simulink model "plant_model_with_dither_input"  (R2024b)
settings: Solver=FixedStepAuto  StartTime=0.0  StopTime=60  FixedStep=T_sample  RelTol=1e-3
values from neighbouring files (symbols this model uses):
  T_sample = 0.01    [LS_demo_ident.m]    (also in P_ident.m)
libraries: simulink x1
settings Model: Creator=Kang  LastModifiedBy=sk3547969879
settings SolverCC: AlgebraicLoopSolver=TrustRegion
settings DebuggingCC: UnconnectedInputMsg=warning  UnconnectedOutputMsg=warning  UnconnectedLineMsg=warning
settings ModelReferenceCC: EnableRefExpFcnMdlSchedulingChecks=on
settings RTWCC: GPUComputeCapability=3.5  DLArmComputeVersion=19.05

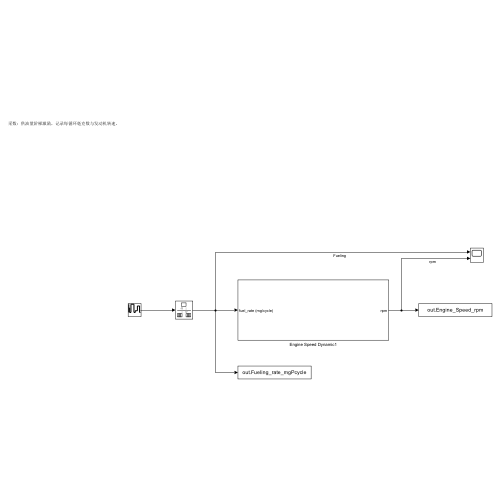
[thumbnail: Simulink's stored preview of the top-level diagram]
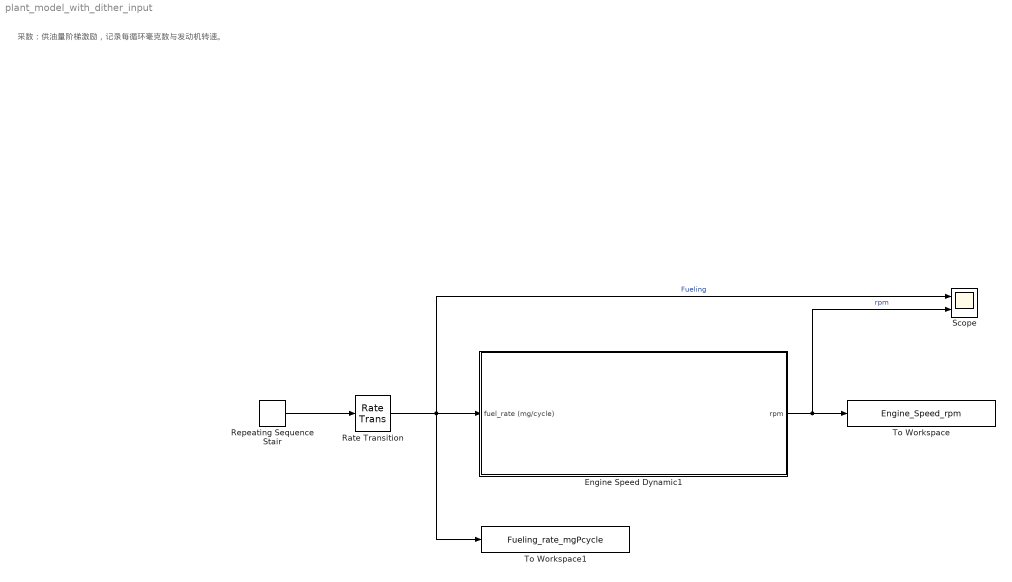
== system plant_model_with_dither_input ==
  note: 采数：供油量阶梯激励，记录每循环毫克数与发动机转速。
  Engine Speed Dynamic1 : Subsystem
  Rate Transition : RateTransition  InitialCondition=10
  Repeating Sequence Stair : simulink/Sources/Repeating Sequence Stair  OutValues=[15 10 20 20 20 10 12 12 18 18 10].'  tsamp=5  OutMin=[]  OutMax=[]  OutDataTypeStr=double  OutputDataTypeScalingMode=double  OutDataType=fixdt(0,8)  ConRadixGroup=Best Precision: Vector-wise  OutScaling=2^-12
  Scope : Scope  NumInputPorts=2
  To Workspace : ToWorkspace  VariableName=Engine_Speed_rpm  SaveFormat=Timeseries  SampleTime=T_sample
  To Workspace1 : ToWorkspace  VariableName=Fueling_rate_mgPcycle  SaveFormat=Timeseries  SampleTime=T_sample
  wires:
  Engine Speed Dynamic1/1(rpm) -> Scope/2, To Workspace/1  "rpm"
  Repeating Sequence Stair/1 -> Rate Transition/1
  Rate Transition/1 -> To Workspace1/1, Scope/1, Engine Speed Dynamic1/1(fuel_rate (mg/cycle))  "Fueling"

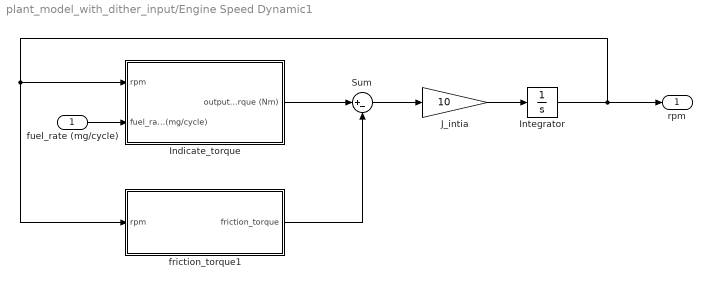
== system plant_model_with_dither_input/Engine Speed Dynamic1 ==
  fuel_rate (mg/cycle) : Inport
  Indicate_torque : Subsystem
  Integrator : Integrator  InitialCondition=960
  J_intia : Gain  Gain=10
  Sum : Sum  Inputs=|+-
  friction_torque1 : Subsystem
  rpm : Outport
  wires:
  Sum/1 -> J_intia/1
  Indicate_torque/1(output_torque (Nm)) -> Sum/1
  Integrator/1 -> rpm/1, friction_torque1/1(rpm), Indicate_torque/1(rpm)
  fuel_rate (mg/cycle)/1 -> Indicate_torque/2(fuel_rate (mg/cycle))
  friction_torque1/1(friction_torque) -> Sum/2
  J_intia/1 -> Integrator/1

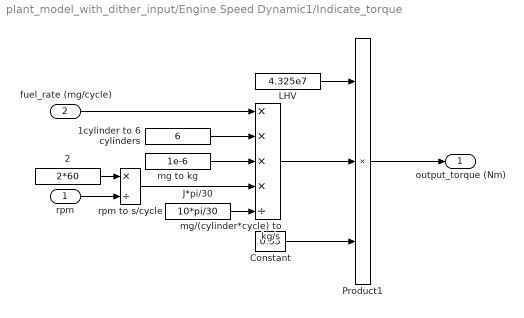
== system plant_model_with_dither_input/Engine Speed Dynamic1/Indicate_torque ==
  rpm : Inport
  fuel_rate (mg/cycle) : Inport  Port=2
  1cylinder to 6 cylinders : Constant  Value=6
  2 : Constant  Value=2*60
  Constant : Constant  Value=0.35
  J*pi/30 : Constant  Value=10*pi/30
  LHV : Constant  Value=4.325e7
  Product1 : Product  Inputs=3
  mg to kg : Constant  Value=1e-6
  mg/(cylinder*cycle) to kg/s : Product  Inputs=****/
  rpm to s/cycle : Product  Inputs=*/
  output_torque (Nm) : Outport
  wires:
  Product1/1 -> output_torque (Nm)/1
  Constant/1 -> Product1/3
  fuel_rate (mg/cycle)/1 -> mg/(cylinder*cycle) to kg/s/1
  1cylinder to 6 cylinders/1 -> mg/(cylinder*cycle) to kg/s/2
  2/1 -> rpm to s/cycle/1
  mg to kg/1 -> mg/(cylinder*cycle) to kg/s/3
  LHV/1 -> Product1/1
  J*pi/30/1 -> mg/(cylinder*cycle) to kg/s/5
  rpm to s/cycle/1 -> mg/(cylinder*cycle) to kg/s/4
  rpm/1 -> rpm to s/cycle/2
  mg/(cylinder*cycle) to kg/s/1 -> Product1/2

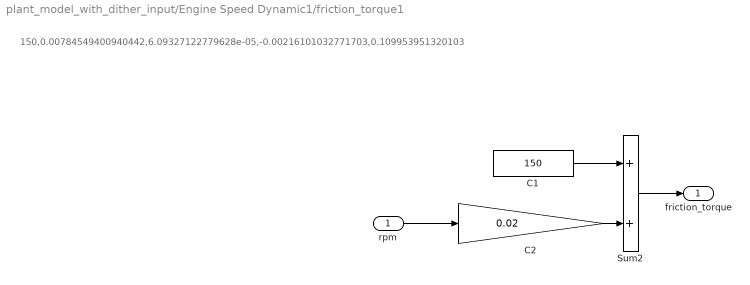
== system plant_model_with_dither_input/Engine Speed Dynamic1/friction_torque1 ==
  note: 150,0.00784549400940442,6.09327122779628e-05,-0.00216101032771703,0.109953951320103
  rpm : Inport
  C1 : Constant  Value=150
  C2 : Gain  Gain=0.02
  Sum2 : Sum
  friction_torque : Outport
  wires:
  rpm/1 -> C2/1
  C1/1 -> Sum2/1
  C2/1 -> Sum2/2
  Sum2/1 -> friction_torque/1
